simulink library "Spring_Control_Hydropneumatic"  (R2025a)
settings: Solver=VariableStepAuto  StartTime=0.0  StopTime=10.0  RelTol=1e-3
libraries: Vehicle_Outputs x1
Description:
  | Copyright 2026 The MathWorks, Inc.
settings Model: Creator=smiller  LastModifiedBy=smiller
settings OptimizationCC: ReuseModelBlockBuffer=off
settings ModelReferenceCC: EnableRefExpFcnMdlSchedulingChecks=on
settings RTWCC: GPUComputeCapability=3.5

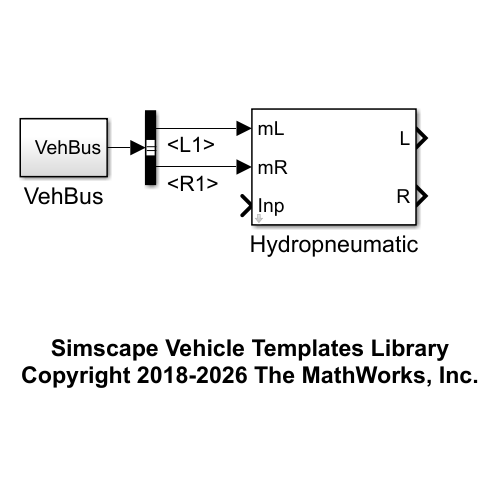
[thumbnail: Simulink's stored preview of the top-level diagram]
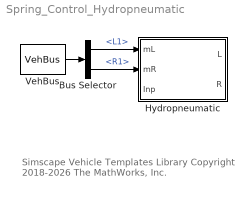
== system Spring_Control_Hydropneumatic ==
  note: Simscape Vehicle Templates Library
      | Copyright 2018-2026 The MathWorks, Inc.
  Bus Selector : BusSelector  OutputSignals=Chassis.Damper.L1,Chassis.Damper.R1
  Hydropneumatic : Subsystem  VariantControl=Choice  mask{popup_gas_spring=Soft}
      mask prompts: popup_gas_spring "Gas Spring"
      mask init:
      | bh = gcb;
      | popup_gas_spring_str = get_param(bh,'popup_gas_spring');
      | 
      | if(strcmp(popup_gas_spring_str,'Stiff'))
      |     soft_suspension = 0;
      | elseif(strcmp(popup_gas_spring_str,'Soft'))
      |     soft_suspension = 1;
      | end
      mask TypeOptions popup_gas_spring: Stiff | Soft
  VehBus : Vehicle_Outputs/VehBus  SystemSampleTime=-1  VariantActivationTime=update diagram  EmptyChoice=off  PassThrough=off  PassThroughVariantControl=(default)  EmptyChoiceVariantControl=(default)  AllowFlexibleInterface=on  Latency=0  AutoFrameSizeCalculation=off
  wires:
  VehBus/1 -> Bus Selector/1
  Bus Selector/1 -> Hydropneumatic/1(mL)  "<L1>"
  Bus Selector/2 -> Hydropneumatic/2(mR)  "<R1>"

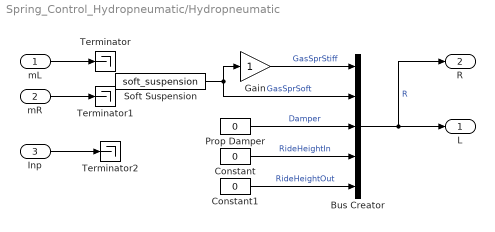
== system Spring_Control_Hydropneumatic/Hydropneumatic ==
  mL : Inport
  mR : Inport  Port=2
  Inp : Inport  Port=3
  Bus Creator : BusCreator  Inputs=5
  Constant : Constant  Value=0
  Constant1 : Constant  Value=0
  Gain : Gain
  Prop Damper : Constant  Value=0
  Soft Suspension : Constant  Value=soft_suspension
  Terminator : Terminator
  Terminator1 : Terminator
  Terminator2 : Terminator
  L : Outport  VectorParamsAs1DForOutWhenUnconnected=off
  R : Outport  Port=2  VectorParamsAs1DForOutWhenUnconnected=off
  wires:
  Constant/1 -> Bus Creator/4  "RideHeightIn"
  Prop Damper/1 -> Bus Creator/3  "Damper"
  Soft Suspension/1 -> Gain/1, Bus Creator/2  "GasSprSoft"
  Gain/1 -> Bus Creator/1  "GasSprStiff"
  Constant1/1 -> Bus Creator/5  "RideHeightOut"
  Inp/1 -> Terminator2/1
  mR/1 -> Terminator1/1
  mL/1 -> Terminator/1
  Bus Creator/1 -> L/1, R/1  "R"
